simulink model "sl_lanechange"  (R2019b)
settings: Solver=ode45  StartTime=0.0  StopTime=10.0  RelTol=1e-3  EnableMultiTasking=on
libraries: simulink x2, roblocks x1
settings Model: Creator=pic  LastModifiedBy=corkep
settings DataIOCC: LimitDataPoints=on  SaveFormat=Array  SignalLoggingSaveFormat=ModelDataLogs  SignalLogging=off  DSMLogging=off  VisualizeSimOutput=off  TimeSaveName=t  OutputSaveName=y
settings OptimizationCC: ExpressionDepthLimit=2147483647  LifeSpan=inf
settings DebuggingCC: UnderspecifiedInitializationDetection=Classic  MergeDetectMultiDrivingBlocksExec=none  SolverPrmCheckMsg=warning  FcnCallInpInsideContextMsg=warning  AllowSymbolicDim=off  StateNameClashWarn=warning  SFUnexpectedBacktrackingDiag=warning  SFNoUnconditionalDefaultTransitionDiag=warning  ArithmeticOperatorsInVariantConditions=warning
settings HardwareCC: ProdBitPerPointer=32  ProdBitPerSizeT=32  ProdBitPerPtrDiffT=32  ProdLargestAtomicFloat=None  ProdIntDivRoundTo=Undefined  ProdEndianess=Unspecified  ProdWordSize=32  ProdHWDeviceType=32-bit Generic
settings ModelReferenceCC: PropagateSignalLabelsOutOfModel=off
settings SFSimCC: SimUseLocalCustomCode=off  CustomCodeUndefinedFunction=UseInterfaceOnly
settings RTWCC: RTWUseLocalCustomCode=off
settings CodeAppCC: StateflowObjectComments=on
settings GRTTargetCC: TargetLangStandard=C89/C90 (ANSI)  GeneratePreprocessorConditionals=Disable all  CombineOutputUpdateFcns=off  GRTInterface=on
settings ConfigComp: CovMetricSettings=dw  CovHtmlReporting=on  CovSaveCumulativeToWorkspaceVar=on  CovSaveSingleToWorkspaceVar=on  CovExternalEMLEnable=off

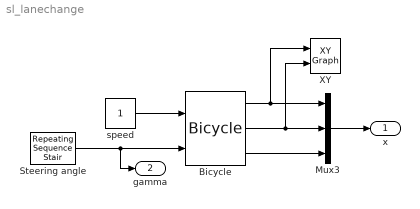
== system sl_lanechange ==
  Bicycle : roblocks/Vehicles/Bicycle  vlim=1  accel=Inf  alim=2  steer_rate=Inf  L=1  x0=[0, 0, 0]
  Mux3 : Mux  Inputs=3
  Steering angle : simulink/Sources/Repeating Sequence Stair  OutValues=[0 0 0 0.5 0 -0.5 0 0 0 0]  tsamp=1  OutMin=[]  OutMax=[]  OutDataTypeStr=double  OutputDataTypeScalingMode=Specify via dialog  OutDataType=double  ConRadixGroup=Best Precision: Vector-wise  OutScaling=2^-12
  XY : simulink/Sinks/XY Graph  xmin=0  xmax=10  ymin=0  ymax=4  st=-1
  speed : Constant  VectorParams1D=off  SampleTime=0.02
  x : Outport
  gamma : Outport  Port=2
  wires:
  Steering angle/1 -> gamma/1, Bicycle/2
  speed/1 -> Bicycle/1
  Bicycle/3 -> Mux3/3
  Bicycle/1 -> Mux3/1, XY/1
  Bicycle/2 -> Mux3/2, XY/2
  Mux3/1 -> x/1
